simulink model "REAL_THREE_TANK"  (R2025b)
settings: Solver=ode15s  StartTime=0.0  StopTime=1500  RelTol=1e-3
InitFcn:
  | run("index.m")
StopFcn:
  | data_name = "realtime_data";
  | save_name = format_file_name(data_name,true);
  | 
  | % Save output data
  | save(save_name,"out")
values from neighbouring files (symbols this model uses):
  adaptParam = 0.15    [index.m]
  hiddenStates = 0    [index.m]
  model_const = struct()    [index.m]
undefined symbols (not defined in the file or in its folder): CR, LF, sigbuilder_block
libraries: instrumentseriallib x3, simulink x1
(part 2 of 2)

== matlab function REAL_THREE_TANK/DR-NMPC/NMPC  ==
  data: uopt output; y_pred output; fcost output size=[1,1]; Ecount output; exitflag output; xPx output; Tconst output; y_set input; ypast input; yo input; tp input; ts input; dist input; upast input; uo input; u_set input; ho input; hk output; modelName input
function [uopt, y_pred, fcost, Ecount, exitflag, xPx, Tconst, hk] = nmpc( y_set, ypast, yo, tp, ts, dist, upast, uo, u_set, ho, modelName)
 % function [uopt, y_pred, fcost, Ecount, exitflag, xPx, Tconst,hk] = nmpc(alpha, y_set, ypast,yo, tp, ts, dist, upast,uo,u_set, ho, modelName ...
    % )

uopt = [0;0;0];
fcost = 0;
y_pred = [0;0;0];

% Regression
u_reg = [upast(1) upast(2), upast(3);uo(1) uo(2),uo(3)];
y_reg =[ypast';yo'];
Ecount = 0 ;
exitflag = Inf ;
xPx = 0 ;
Tconst = 0 ;
hk = ho;
% Steady states

h1ss=y_set(1) ; h2ss=y_set(2) ; h3ss=y_set(3) ; 
u1ss=u_set(1) ; u2ss=u_set(2) ; u3ss = u_set(3);
% h1ss=14.6 ; h2ss=18.15 ; h3ss=17.7 ; 
% u1ss=130 ; u2ss=0.4 ; u3ss = 0.2;

%  
% rhoux = 10;
% rhou = 5;
% from DR
rhoux = 20;
rhou = 1;
% 
Wy = [1/h1ss, 1/h2ss, 1/h3ss]*rhoux;
% Wy = [2/h1ss, 1/h2ss, 2/h3ss, 1/h4ss];
% Wy = [0.5, 0.5, 0.5];
Wu =  [1/u1ss,1/u2ss, 1/u3ss]*rhou;
% Wu =  [0.15,0.15];
% Wdu = [1/u1ss,1/u2ss, 1/u3ss]*5;
Wdu =[0.075, 1000, 1000];
Wuerr=[1/u1ss,1/u2ss, 1/u3ss]*rhou;

P1 = [
    0.3408    0.1535    0.0676;
    0.1535    0.4748    0.2177;
    0.0676    0.2177    0.6235;
    ];

alpha1 = 262.0298;
K1 =[
    0.2349    0.0934    0.0358;
    0.1045    0.1734    0.0648;
    0.0366    0.0650    0.1542;];

P2 =[
    0.3369    0.1626    0.0659;
    0.1626    0.6218    0.3412;
    0.0659    0.3412    0.6925;
    ];
alpha2 =19.4123;

P3 =[
    0.3408    0.1556    0.0754;
    0.1556    0.4888    0.2504;
    0.0754    0.2504    0.6810;];
alpha3 = 20.4206;

P4 = [
    0.3137    0.0167    0.0102;
    0.0167    0.1433    0.0367;
    0.0102    0.0367    0.1221;
    ] ; %dlqr
alpha4 = 14.0453;

% From DR
P5 =[5.8219    0.2246    0.1820
    0.2246    2.1818    0.4469
    0.1820    0.4469    2.0162] ;


K5 = [0.8819    0.0450    0.0292
   -0.0183   -0.0858    0.0248
   -0.0113   -0.0404   -0.0658] ;

alpha5=16.1835;
% 
P=P3;
alpha = alpha1;


nu = tp(1);
ny = tp(2);
Nu = tp(3);
Np = tp(4);

bounds = struct();
% bounds.ymin =[0.1 ,0.1, 0.1];
% bounds.ymax =[30 30 30];
% bounds.u_min = [0.1 0.1 0.1];
% bounds.u_max = [250, 1, 1];
bounds.ymin =[0 ,0, 0];
bounds.ymax =[35 35 35];
bounds.u_min = [0 0 0];
bounds.u_max = [200, 1, 1];
% du = [50, 0.25, 0.25];
du = [20, 0.1, 0.1];
bounds.du_min =  -du;
bounds.du_max = du;

% bounds.du_min =  -2*ones(1, nu);
% bounds.du_max = 2*ones(1, nu);
params = struct();
params.y_set = y_set;
params.u_set = u_set;
params.nu = nu;
params.ny = ny;
params.Nu = Nu;
params.Np = Np;
params.Wy = Wy;
params.Wdu = Wdu;
params.Wu = Wu;
params.Wuerr =Wuerr;
params.ts = ts;
params.P = P;
params.alpha = alpha;
params.modelName = modelName;
params.bounds = bounds;
params.dist = dist;

coder.extrinsic('get_control_input');


[uopt, y_pred, hk, fval, exitflag, elapsed, ~, ~] = get_control_input(y_reg, u_reg, ho, params);
% uopt = uk;
% y_pred = yk;
% info = [ fval,exitflag, elapsed, xPx, Tconst, uopt];
% 
fcost = fval;
Ecount = elapsed ;
exitflag = exitflag ;
% xPx = xPx ;
% Tconst = Tconst ;
end

== matlab function REAL_THREE_TANK/Disturbance Rejector ==
  data: r_k input; dist output; y_plant input; W_dist input; dist_old input
function dist = Dist_rejector(r_k, y_plant, W_dist, dist_old)
% DIST_REJECTOR: integral-type disturbance estimate for offset-free NMPC
%   dist_k = dist_{k-1} + W_dist * (y_k - r_k)
%
% Changes from the original:
%   1. Linear error instead of tanh(e). tanh saturated at |e| > ~2 cm, which
%      capped the update at W_dist per step and made large disturbances
%      recover along a slow straight line.
%   2. Anti-windup: integration is frozen for FREEZE_STEPS samples after any
%      setpoint change, so servo steps (large but expected tracking error)
%      do not wind the estimate up.
%   3. Estimate clamped to +/- D_MAX.
%
% Inputs:
%   r_k      - setpoint [3x1]
%   y_plant  - measured levels [3x1]
%   W_dist   - integration gain (scalar or [3x1])
%   dist_old - previous estimate [3x1]

FREEZE_STEPS = 30;   % 30 samples = 60 s at Ts = 2 s
D_MAX        = 15;   % cm

persistent r_prev hold_cnt
if isempty(r_prev)
    r_prev   = r_k;
    hold_cnt = 0;
end

% setpoint changed -> start freeze
if any(abs(r_k(:) - r_prev(:)) > 1e-6)
    hold_cnt = FREEZE_STEPS;
end
r_prev = r_k;

e_k = y_plant - r_k;

if hold_cnt > 0
    hold_cnt = hold_cnt - 1;
    dist = dist_old;                    % frozen
else
    dist = dist_old + W_dist .* e_k;    % linear integral update
end

dist = min(max(dist, -D_MAX), D_MAX);
end


% function dist = Dist_rejector(r_k, y_plant, W_dist, dist_old)
% % DIST_REJECTOR: Estimates disturbance based on output error
% %
% % Inputs:
% %   r_k      - Reference/predicted output (scalar or array)
% %   y_plant  - Actual plant output (scalar or array)
% %   W_dist   - Disturbance gain (scalar or array)
% %   dist_old - Previous disturbance estimate (scalar or array)
% %
% % Output:
% %   dist     - Updated disturbance estimate (same size as r_k)
%     % Compute element-wise error
%     % disp(size(r_k))
%     %   disp(size(y_plant))
%     %   disp(size(dist_old))
%     e_k = y_plant - r_k;
% 
%     % Permissible error bounds (change if needed)
%     error_min = -Inf;
%     error_max =  Inf;
% 
%     % Apply tanh only within bounds
%     valid_mask = (e_k > error_min) & (e_k < error_max);
%     error_func = zeros(size(e_k), 'like', e_k);
%     error_func(valid_mask) = tanh(e_k(valid_mask));
%     % Alternative: error_func(valid_mask) = e_k(valid_mask);
% 
%     % Element-wise disturbance update
%     dist = error_func .* W_dist + dist_old;
% end

== matlab function REAL_THREE_TANK/Three tank sys/THREE_TANKS REALTIME_ PLANT/3 TANK  SYSTEM /SEND/MATLAB Function2 ==
  data: real_ht input; y output; set_ht input; set_min input; Valvm_in input
function y = fcn(real_ht,set_ht,set_min,Valvm_in)
      temp = Valvm_in;
if (real_ht >= set_ht)
      temp = set_min;
 end
       
y = temp;

== matlab function REAL_THREE_TANK/Three tank sys/THREE_TANKS REALTIME_ PLANT/3 TANK  SYSTEM /SEND/MATLAB Function ==
  data: s input; a input; y output; b input; c input; d input; e input; f input
function y = fcn(s,a,b,c,d,e,f) %,power,rst)
% persistent a_;
% persistent b_;
% persistent c_;
% persistent d_;
% persistent e_;
% if (power == 1)
 temp = [s,a,b,c,d,e,f];
% end   

% if (power == 0)
%  temp =  rst %[0,0,0,0,0]
% end

y = temp;
